simulink model "AEB_S1"  (R2024a)
settings: Solver=ode45  StartTime=0.0  StopTime=10  FixedStep=0.0001  MaxStep=0.01  RelTol=1e-3
libraries: Solver_SF x1
settings Model: Creator=HP  LastModifiedBy=HP

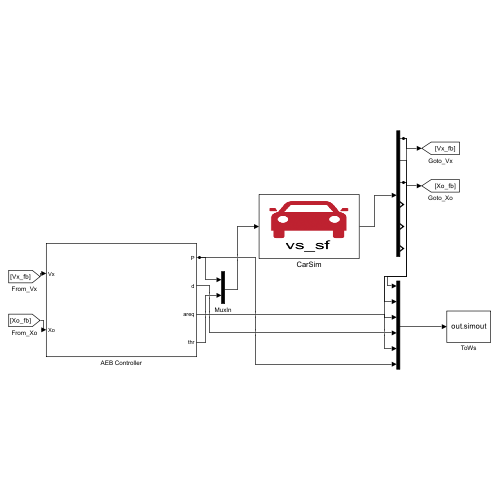
[thumbnail: Simulink's stored preview of the top-level diagram]
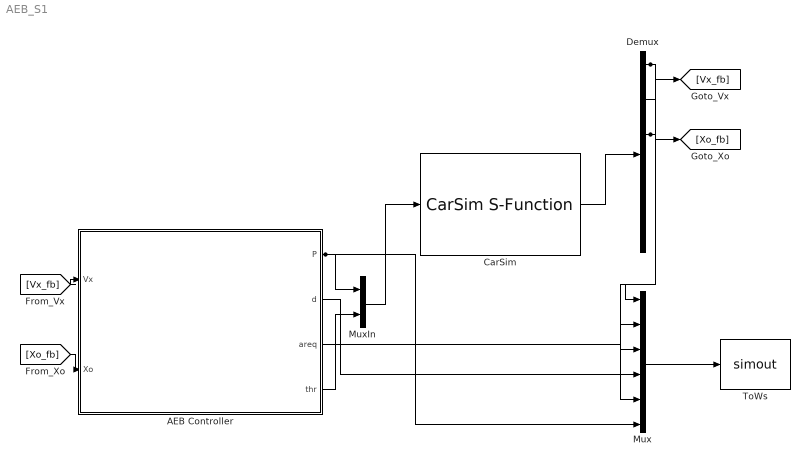
== system AEB_S1 ==
  AEB Controller : Subsystem
  CarSim : Solver_SF/CarSim S-Function  Priority=1  SIMFILE=E:\carsim2024data1\simfile.sim  Run_RTs=off  vs_state_ind=Run  StopMode_ind=Vehicle Model
  Demux : Demux  Outputs=6
  Mux : Mux  Inputs=6
  MuxIn : Mux  Inputs=2
  ToWs : ToWorkspace  VariableName=simout  SaveFormat=Structure With Time  SampleTime=-1
  wires:
  [Vx_fb] -> AEB Controller/1(Vx)
  [Xo_fb] -> AEB Controller/2(Xo)
  AEB Controller/1(P) -> MuxIn/1, Mux/6
  AEB Controller/4(thr) -> MuxIn/2
  MuxIn/1 -> CarSim/1
  CarSim/1 -> Demux/1
  Demux/1 -> [Vx_fb], Mux/1
  Demux/3 -> [Xo_fb], Mux/3
  Demux/2 -> Mux/2
  AEB Controller/2(d) -> Mux/4
  AEB Controller/3(areq) -> Mux/5
  Mux/1 -> ToWs/1

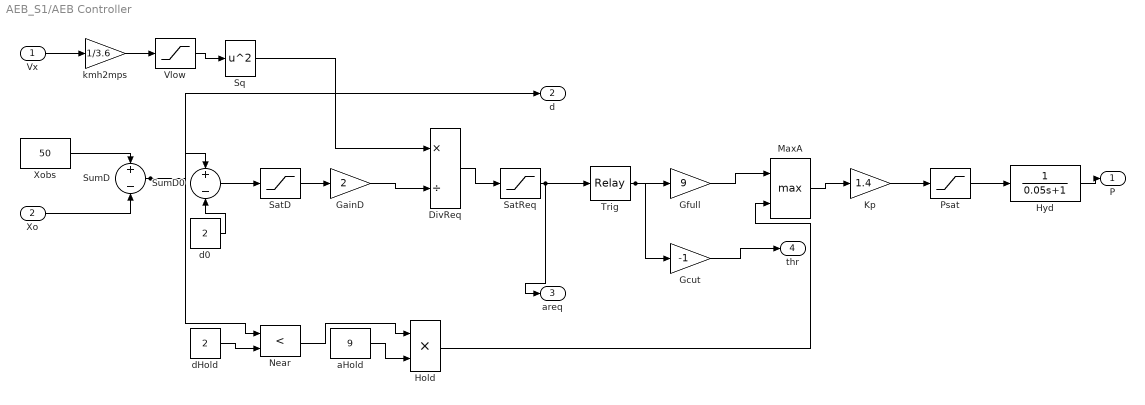
== system AEB_S1/AEB Controller ==
  Vx : Inport
  Xo : Inport  Port=2
  DivReq : Product  Inputs=*/
  GainD : Gain  Gain=2
  Gcut : Gain  Gain=-1
  Gfull : Gain  Gain=9
  Hold : Product
  Hyd : TransferFcn  Denominator=[0.05 1]
  Kp : Gain  Gain=1.4
  MaxA : MinMax  Function=max  Inputs=2
  Near : RelationalOperator  Operator=<  OutDataTypeStr=boolean  RndMeth=Simplest  InputSameDT=off
  Psat : Saturate  UpperLimit=14  LowerLimit=0
  SatD : Saturate  UpperLimit=inf  LowerLimit=0.5
  SatReq : Saturate  UpperLimit=9  LowerLimit=0
  Sq : Math  Operator=square
  SumD : Sum  Inputs=+-
  SumD0 : Sum  Inputs=+-
  Trig : Relay  OnSwitchValue=5  OffSwitchValue=-1
  Vlow : Saturate  UpperLimit=inf  LowerLimit=0.5
  Xobs : Constant  Value=50
  aHold : Constant  Value=9
  d0 : Constant  Value=2
  dHold : Constant  Value=2
  kmh2mps : Gain  Gain=1/3.6
  P : Outport
  d : Outport  Port=2
  areq : Outport  Port=3
  thr : Outport  Port=4
  wires:
  Vx/1 -> kmh2mps/1
  kmh2mps/1 -> Vlow/1
  Vlow/1 -> Sq/1
  Xobs/1 -> SumD/1
  Xo/1 -> SumD/2
  SumD/1 -> SumD0/1, Near/1, d/1
  d0/1 -> SumD0/2
  SumD0/1 -> SatD/1
  SatD/1 -> GainD/1
  Sq/1 -> DivReq/1
  GainD/1 -> DivReq/2
  DivReq/1 -> SatReq/1
  SatReq/1 -> Trig/1, areq/1
  Trig/1 -> Gfull/1, Gcut/1
  Gcut/1 -> thr/1
  dHold/1 -> Near/2
  Near/1 -> Hold/1
  aHold/1 -> Hold/2
  Gfull/1 -> MaxA/1
  Hold/1 -> MaxA/2
  MaxA/1 -> Kp/1
  Kp/1 -> Psat/1
  Psat/1 -> Hyd/1
  Hyd/1 -> P/1
